simulink model "FinalSolution_2025ElectricalComp"  (R2025b)
settings: Solver=VariableStepAuto  StartTime=0.0  StopTime=0.8  FixedStep=SPWM_Ts  RelTol=1e-3
InitFcn:
  | evalin(get_param(bdroot,'ModelWorkspace'),'eval(VF_InitializeCode);');
model workspace (MAT data in the model file):
  AC_LoadResistance = 9.23760430703
  AD_TimeConstant = 0.00025
  AD_a = [1 -0.881765205117]
  AD_b = [2.95586987209 -2.95586987209]
  CL_AAComp = 1.00249999972
  CL_AA_a = 0.998744152176
  CL_Kaw = 20
  CL_Ki = 1.6
  CL_Kp = 0.005
  CL_N = 200
  CL_Ts = 0.0001
  CL_Vref = 32
  CL_faa = 1000
  CL_fp = 50
  CL_mff = 0.94
  CL_mmax = 1
  CommonModeBias = 0.15
  CommonModeKp = 0.02
  CommonModeShift = 1
  ControlStartTime = 0.06
  DampingCapuF = 4.7
  DampingResistance = 30
  DeadtimeComp = 0.08
  DeadtimeCurrentBand = 0.2
  DutyFeedforward = 0
  DutyMax = 0.75
  FilterDCR = 0.3
  KiCurrentLoop = 5
  KiVoltageLoop = 5
  KpCurrentLoop = 0.08
  KpVoltageLoop = 0.2
  LoadConnectTime = 0.18
  MainFilterCapuF = 4.7
  PR_Gain = 1.25
  PR_a10 = [1 -1.99838562653 0.999372033695]
  PR_a11 = [1 -1.99817857535 0.999372066214]
  PR_a13 = [1 -1.99770539603 0.999372140529]
  PR_a16 = [1 -1.99684804391 0.99937227518]
  PR_a17 = [1 -1.99652293757 0.99937232624]
  PR_a19 = [1 -1.9958137982 0.999372437614]
  PR_a2 = [1 -1.99933241937 0.999371884997]
  PR_a4 = [1 -1.99921404574 0.999371903588]
  PR_a5 = [1 -1.99912527012 0.99937191753]
  PR_a7 = [1 -1.9988885544 0.999371954708]
  PR_a8 = [1 -1.99874062131 0.999371977941]
  PR_b10 = [0.236875635534 -0.472442728614 0.23556709308]
  PR_b11 = [0.215389811794 -0.429471148895 0.214081337101]
  PR_b13 = [0.182331988259 -0.363355656682 0.181023668423]
  PR_b16 = [0.148235597863 -0.295163156474 0.146927558611]
  PR_b17 = [0.139542977111 -0.277778021366 0.138235044255]
  PR_b19 = [0.124900915012 -0.248494129248 0.123593214235]
  PR_b2 = [0.425928775502 -0.847596177142 0.42166740164]
  PR_b4 = [0.279572378961 -0.55553023994 0.275957860979]
  PR_b5 = [0.246657018631 -0.490084248228 0.243427229597]
  PR_b7 = [0.202908225742 -0.403457656245 0.200549430503]
  PR_b8 = [0.186290317354 -0.370698545076 0.184408227722]
  PrechargeBypassTime = 0.16
  PrechargeResistance = 47
  RegenerativeMode = 1
  ReturnCurrent = 1.5
  ReturnRampTime = 0.08
  ReturnTs = 1e-05
  Return_Iref = 2
  SPWM_Ndead = 10
  SPWM_Tdead = 2e-06
  SPWM_Ts = 2e-07
  SPWM_Vgate = 10
  SPWM_f1 = 50
  SPWM_fs = 20000
  SPWM_m = 0.8
  Test_Mode = 1
  VF_CurrentN = 2000
  VF_CurrentRampTime = 0.1
  VF_InitializeCode : object (value not decoded)
  VF_LoadR = 9.23760430703
  VF_PR_Analog50 : object (value not decoded)
  VF_PR_Base50 : object (value not decoded)
  VF_ReturnStart = 0.08
  VF_mff32 = 0.94
  VoltageRampRate = 100
  op_snapshot1 : opcond.OperatingPoint (value not decoded)
  testadd = 0
undefined symbols (not defined in the file): DiscIntNeverNeededParam, dspblkCoreblockFVToolHelper, gcbh
libraries: fl_lib x37, ee_lib x37, nesl_utility x32
(part 4 of 4)

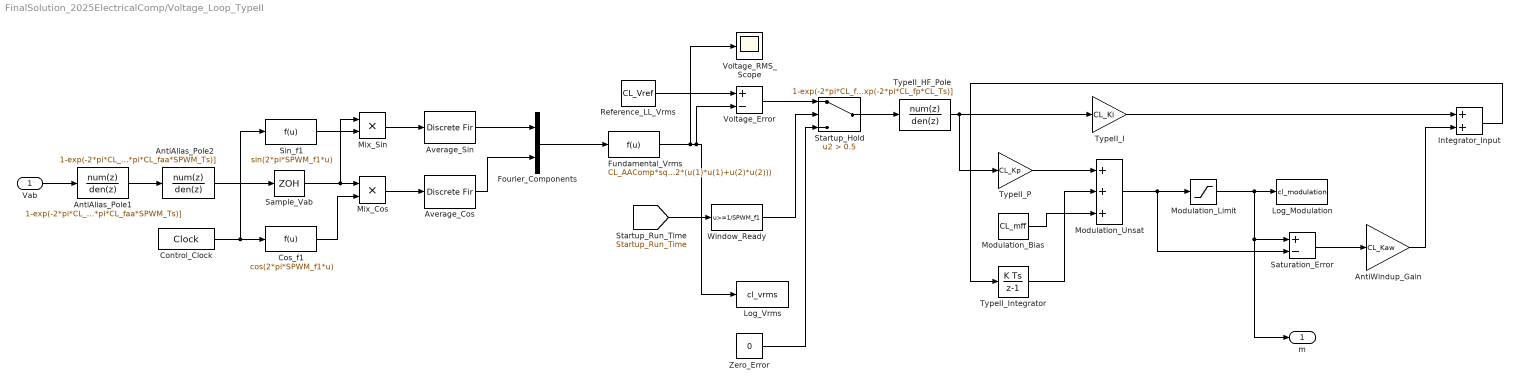
== system FinalSolution_2025ElectricalComp/Voltage_Loop_TypeII ==
  Vab : Inport
  AntiAlias_Pole1 : DiscreteTransferFcn  LoadFcn=dspblkCoreblockFVToolHelper(gcbh,'load');  Numerator=1-exp(-2*pi*CL_faa*SPWM_Ts)  Denominator=[1 -exp(-2*pi*CL_faa*SPWM_Ts)]  SampleTime=SPWM_Ts
      settings: CopyFcn=dspblkCoreblockFVToolHelper(gcbh,'copy');  DeleteFcn=dspblkCoreblockFVToolHelper(gcbh,'close');  ModelCloseFcn=dspblkCoreblockFVToolHelper(gcbh,'close');  PreSaveFcn=dspblkCoreblockFVToolHelper(gcbh,'presave');  PostSaveFcn=dspblkCoreblockFVToolHelper(gcbh,'postsave');  CloseFcn=dspblkCoreblockFVToolHelper(gcbh,'close');
  AntiAlias_Pole2 : DiscreteTransferFcn  LoadFcn=dspblkCoreblockFVToolHelper(gcbh,'load');  Numerator=1-exp(-2*pi*CL_faa*SPWM_Ts)  Denominator=[1 -exp(-2*pi*CL_faa*SPWM_Ts)]  SampleTime=SPWM_Ts
      settings: CopyFcn=dspblkCoreblockFVToolHelper(gcbh,'copy');  DeleteFcn=dspblkCoreblockFVToolHelper(gcbh,'close');  ModelCloseFcn=dspblkCoreblockFVToolHelper(gcbh,'close');  PreSaveFcn=dspblkCoreblockFVToolHelper(gcbh,'presave');  PostSaveFcn=dspblkCoreblockFVToolHelper(gcbh,'postsave');  CloseFcn=dspblkCoreblockFVToolHelper(gcbh,'close');
  AntiWindup_Gain : Gain  Gain=CL_Kaw
  Average_Cos : DiscreteFir  LoadFcn=dspblkCoreblockFVToolHelper(gcbh,'load');  Coefficients=ones(1,CL_N)/CL_N  SampleTime=CL_Ts
      settings: CopyFcn=dspblkCoreblockFVToolHelper(gcbh,'copy');  DeleteFcn=dspblkCoreblockFVToolHelper(gcbh,'close');  ModelCloseFcn=dspblkCoreblockFVToolHelper(gcbh,'close');  PreSaveFcn=dspblkCoreblockFVToolHelper(gcbh,'presave');  PostSaveFcn=dspblkCoreblockFVToolHelper(gcbh,'postsave');  CloseFcn=dspblkCoreblockFVToolHelper(gcbh,'close');
  Average_Sin : DiscreteFir  Coefficients=ones(1,CL_N)/CL_N  SampleTime=CL_Ts
  Control_Clock : DigitalClock  SampleTime=CL_Ts
  Cos_f1 : Fcn  Expr=cos(2*pi*SPWM_f1*u)
  Fourier_Components : Mux  Inputs=2
  Fundamental_Vrms : Fcn  Expr=CL_AAComp*sqrt(2*(u(1)*u(1)+u(2)*u(2)))
  Integrator_Input : Sum
  Log_Modulation : ToWorkspace  VariableName=cl_modulation  SaveFormat=Timeseries  SampleTime=CL_Ts
  Log_Vrms : ToWorkspace  VariableName=cl_vrms  SaveFormat=Timeseries  SampleTime=CL_Ts
  Mix_Cos : Product
  Mix_Sin : Product
  Modulation_Bias : Constant  Value=CL_mff
  Modulation_Limit : Saturate  UpperLimit=CL_mmax  LowerLimit=0
  Modulation_Unsat : Sum  Inputs=+++
  Reference_LL_Vrms : Constant  Value=CL_Vref
  Sample_Vab : ZeroOrderHold  SampleTime=CL_Ts
  Saturation_Error : Sum  Inputs=+-
  Sin_f1 : Fcn  Expr=sin(2*pi*SPWM_f1*u)
  Startup_Hold : Switch  Criteria=u2 > Threshold  Threshold=0.5  SaturateOnIntegerOverflow=off  InputSameDT=off
  TypeII_HF_Pole : DiscreteTransferFcn  LoadFcn=dspblkCoreblockFVToolHelper(gcbh,'load');  Numerator=1-exp(-2*pi*CL_fp*CL_Ts)  Denominator=[1 -exp(-2*pi*CL_fp*CL_Ts)]  SampleTime=CL_Ts
      settings: CopyFcn=dspblkCoreblockFVToolHelper(gcbh,'copy');  DeleteFcn=dspblkCoreblockFVToolHelper(gcbh,'close');  ModelCloseFcn=dspblkCoreblockFVToolHelper(gcbh,'close');  PreSaveFcn=dspblkCoreblockFVToolHelper(gcbh,'presave');  PostSaveFcn=dspblkCoreblockFVToolHelper(gcbh,'postsave');  CloseFcn=dspblkCoreblockFVToolHelper(gcbh,'close');
  TypeII_I : Gain  Gain=CL_Ki
  TypeII_Integrator : DiscreteIntegrator  SampleTime=CL_Ts  ICPrevOutput=DiscIntNeverNeededParam  ICPrevScaledInput=DiscIntNeverNeededParam
  TypeII_P : Gain  Gain=CL_Kp
  Voltage_Error : Sum  Inputs=+-
  Voltage_RMS_Scope : Scope
      settings: TimeSpan=0.45  ActiveDisplayYMinimum=0  ActiveDisplayYMaximum=36
  Window_Ready : Fcn  Expr=u>=1/SPWM_f1
  Zero_Error : Constant  Value=0
  m : Outport
  wires:
  AntiAlias_Pole2/1 -> Sample_Vab/1
  AntiAlias_Pole1/1 -> AntiAlias_Pole2/1
  Vab/1 -> AntiAlias_Pole1/1
  Fundamental_Vrms/1 -> Log_Vrms/1, Voltage_Error/2, Voltage_RMS_Scope/1
  Mix_Sin/1 -> Average_Sin/1
  Cos_f1/1 -> Mix_Cos/2
  Control_Clock/1 -> Sin_f1/1, Cos_f1/1
  Sample_Vab/1 -> Mix_Sin/1, Mix_Cos/1
  TypeII_HF_Pole/1 -> TypeII_P/1, TypeII_I/1
  Sin_f1/1 -> Mix_Sin/2
  Integrator_Input/1 -> TypeII_Integrator/1
  Average_Sin/1 -> Fourier_Components/1
  Mix_Cos/1 -> Average_Cos/1
  Average_Cos/1 -> Fourier_Components/2
  Fourier_Components/1 -> Fundamental_Vrms/1
  Reference_LL_Vrms/1 -> Voltage_Error/1
  Saturation_Error/1 -> AntiWindup_Gain/1
  TypeII_P/1 -> Modulation_Unsat/1
  Modulation_Bias/1 -> Modulation_Unsat/3
  TypeII_Integrator/1 -> Modulation_Unsat/2
  Modulation_Unsat/1 -> Saturation_Error/2, Modulation_Limit/1
  TypeII_I/1 -> Integrator_Input/1
  Modulation_Limit/1 -> m/1, Saturation_Error/1, Log_Modulation/1
  AntiWindup_Gain/1 -> Integrator_Input/2
  [Startup_Run_Time] -> Window_Ready/1
  Startup_Hold/1 -> TypeII_HF_Pole/1
  Zero_Error/1 -> Startup_Hold/3
  Voltage_Error/1 -> Startup_Hold/1
  Window_Ready/1 -> Startup_Hold/2

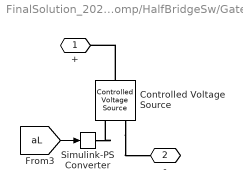
== system FinalSolution_2025ElectricalComp/HalfBridgeSw/GateDri ==
  Controlled Voltage Source : fl_lib/Electrical/Electrical Sources/Controlled Voltage Source
  Simulink-PS Converter : nesl_utility/Simulink-PS Converter  PhysicalDomain=network_engine_domain  SubClassName=ps_input  LeftPortType=input  RightPortType=output  PseudoPeriodic=off  Frequencies=[]  NoiseDistribution=none  NoiseParameters=[]  Unit=1  AffineConversion=off  FilteringAndDerivatives=provide  SimscapeFilterOrder=1  InputFilterTimeConstant=0.001  UdotUserProvided=0
  + : PMIOPort  Side=Left
  - : PMIOPort  Port=2  Side=Right
  wires:
  [aL] -> Simulink-PS Converter/1
  connections:
  Controlled Voltage Source/LConn1 -- +/RConn1
  Simulink-PS Converter/RConn1 -- Controlled Voltage Source/RConn1
  Controlled Voltage Source/RConn2 -- -/RConn1

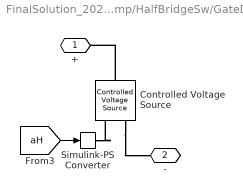
== system FinalSolution_2025ElectricalComp/HalfBridgeSw/GateDri1 ==
  Controlled Voltage Source : fl_lib/Electrical/Electrical Sources/Controlled Voltage Source
  Simulink-PS Converter : nesl_utility/Simulink-PS Converter  PhysicalDomain=network_engine_domain  SubClassName=ps_input  LeftPortType=input  RightPortType=output  PseudoPeriodic=off  Frequencies=[]  NoiseDistribution=none  NoiseParameters=[]  Unit=1  AffineConversion=off  FilteringAndDerivatives=provide  SimscapeFilterOrder=1  InputFilterTimeConstant=0.001  UdotUserProvided=0
  + : PMIOPort  Side=Left
  - : PMIOPort  Port=2  Side=Right
  wires:
  [aH] -> Simulink-PS Converter/1
  connections:
  Controlled Voltage Source/RConn2 -- -/RConn1
  Simulink-PS Converter/RConn1 -- Controlled Voltage Source/RConn1
  Controlled Voltage Source/LConn1 -- +/RConn1

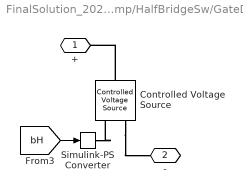
== system FinalSolution_2025ElectricalComp/HalfBridgeSw/GateDri2 ==
  Controlled Voltage Source : fl_lib/Electrical/Electrical Sources/Controlled Voltage Source
  Simulink-PS Converter : nesl_utility/Simulink-PS Converter  PhysicalDomain=network_engine_domain  SubClassName=ps_input  LeftPortType=input  RightPortType=output  PseudoPeriodic=off  Frequencies=[]  NoiseDistribution=none  NoiseParameters=[]  Unit=1  AffineConversion=off  FilteringAndDerivatives=provide  SimscapeFilterOrder=1  InputFilterTimeConstant=0.001  UdotUserProvided=0
  + : PMIOPort  Side=Left
  - : PMIOPort  Port=2  Side=Right
  wires:
  [bH] -> Simulink-PS Converter/1
  connections:
  Controlled Voltage Source/LConn1 -- +/RConn1
  Simulink-PS Converter/RConn1 -- Controlled Voltage Source/RConn1
  Controlled Voltage Source/RConn2 -- -/RConn1

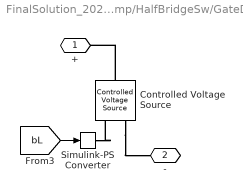
== system FinalSolution_2025ElectricalComp/HalfBridgeSw/GateDri3 ==
  Controlled Voltage Source : fl_lib/Electrical/Electrical Sources/Controlled Voltage Source
  Simulink-PS Converter : nesl_utility/Simulink-PS Converter  PhysicalDomain=network_engine_domain  SubClassName=ps_input  LeftPortType=input  RightPortType=output  PseudoPeriodic=off  Frequencies=[]  NoiseDistribution=none  NoiseParameters=[]  Unit=1  AffineConversion=off  FilteringAndDerivatives=provide  SimscapeFilterOrder=1  InputFilterTimeConstant=0.001  UdotUserProvided=0
  + : PMIOPort  Side=Left
  - : PMIOPort  Port=2  Side=Right
  wires:
  [bL] -> Simulink-PS Converter/1
  connections:
  Controlled Voltage Source/RConn2 -- -/RConn1
  Simulink-PS Converter/RConn1 -- Controlled Voltage Source/RConn1
  Controlled Voltage Source/LConn1 -- +/RConn1

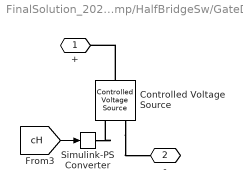
== system FinalSolution_2025ElectricalComp/HalfBridgeSw/GateDri4 ==
  Controlled Voltage Source : fl_lib/Electrical/Electrical Sources/Controlled Voltage Source
  Simulink-PS Converter : nesl_utility/Simulink-PS Converter  PhysicalDomain=network_engine_domain  SubClassName=ps_input  LeftPortType=input  RightPortType=output  PseudoPeriodic=off  Frequencies=[]  NoiseDistribution=none  NoiseParameters=[]  Unit=1  AffineConversion=off  FilteringAndDerivatives=provide  SimscapeFilterOrder=1  InputFilterTimeConstant=0.001  UdotUserProvided=0
  + : PMIOPort  Side=Left
  - : PMIOPort  Port=2  Side=Right
  wires:
  [cH] -> Simulink-PS Converter/1
  connections:
  Controlled Voltage Source/RConn2 -- -/RConn1
  Simulink-PS Converter/RConn1 -- Controlled Voltage Source/RConn1
  Controlled Voltage Source/LConn1 -- +/RConn1

== system FinalSolution_2025ElectricalComp/HalfBridgeSw/GateDri5 ==
  Controlled Voltage Source : fl_lib/Electrical/Electrical Sources/Controlled Voltage Source
  Simulink-PS Converter : nesl_utility/Simulink-PS Converter  PhysicalDomain=network_engine_domain  SubClassName=ps_input  LeftPortType=input  RightPortType=output  PseudoPeriodic=off  Frequencies=[]  NoiseDistribution=none  NoiseParameters=[]  Unit=1  AffineConversion=off  FilteringAndDerivatives=provide  SimscapeFilterOrder=1  InputFilterTimeConstant=0.001  UdotUserProvided=0
  + : PMIOPort  Side=Left
  - : PMIOPort  Port=2  Side=Right
  wires:
  [cL] -> Simulink-PS Converter/1
  connections:
  Controlled Voltage Source/LConn1 -- +/RConn1
  Simulink-PS Converter/RConn1 -- Controlled Voltage Source/RConn1
  Controlled Voltage Source/RConn2 -- -/RConn1
